simulink model "APFv2_alpha"  (R2025a)
settings: Solver=ode45  StartTime=0.0  StopTime=1  RelTol=1e-3  EnableMultiTasking=on
undefined symbols (not defined in the file): Newton, R_nl, Raphson
libraries: spsDiodeLib x12, spsCurrentMeasurementLib x9, spsSeriesRLCBranchLib x9, spsGroundLib x8, spsVoltageMeasurementLib x5, spsACCurrentSourceLib x3, spsThreePhaseBreakerLib x3, spsThreePhaseSeriesRLCBranchLib x3, spsThreePhaseVIMeasurementLib x2, spsThreePhaseSourceLib x1, powerlib_extras x1, dspfdesign x1
settings Model: Creator=Jawad  LastModifiedBy=SimuVerity Contributors
settings SolverCC: AlgebraicLoopSolver=TrustRegion
settings DataIOCC: LimitDataPoints=on  SaveFormat=Array  SignalLoggingSaveFormat=ModelDataLogs  ReturnWorkspaceOutputs=off
settings OptimizationCC: ExpressionDepthLimit=2147483647.0  LifeSpan=inf
settings DebuggingCC: UnderspecifiedInitializationDetection=Classic  MergeDetectMultiDrivingBlocksExec=none  SolverPrmCheckMsg=warning  FcnCallInpInsideContextMsg=warning  UnconnectedInputMsg=warning  UnconnectedOutputMsg=warning  UnconnectedLineMsg=warning  StateNameClashWarn=warning  SFUnexpectedBacktrackingDiag=warning  SFNoUnconditionalDefaultTransitionDiag=warning  SFExecutionAtInitializationDiag=none  ArithmeticOperatorsInVariantConditions=warning
settings HardwareCC: ProdBitPerPointer=32.0  ProdBitPerSizeT=32.0  ProdBitPerPtrDiffT=32.0  ProdLargestAtomicFloat=None  ProdIntDivRoundTo=Undefined  ProdEndianess=Unspecified  ProdWordSize=32.0  ProdHWDeviceType=32-bit Generic
settings ModelReferenceCC: PropagateSignalLabelsOutOfModel=off
settings SFSimCC: SFSimEcho=off  SimUseLocalCustomCode=off  SimParseCustomCode=off  CustomCodeUndefinedFunction=UseInterfaceOnly
settings RTWCC: RTWUseLocalCustomCode=off  GPUComputeCapability=3.5
settings CodeAppCC: StateflowObjectComments=on
settings GRTTargetCC: TargetLangStandard=C89/C90 (ANSI)  CombineOutputUpdateFcns=off  GRTInterface=on
settings ConfigComp: CovMetricSettings=dw  CovSaveCumulativeToWorkspaceVar=on  CovSaveSingleToWorkspaceVar=on  CovExternalEMLEnable=off

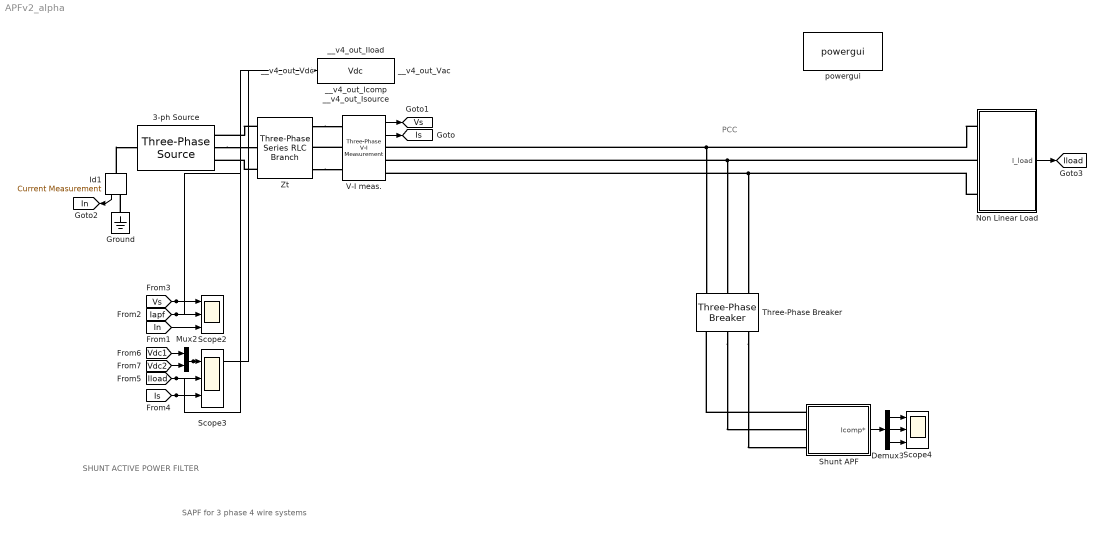
== system APFv2_alpha ==
  note: SHUNT ACTIVE POWER FILTER
  note: PCC
  note: SAPF for 3 phase 4 wire systems
  3-ph Source : spsThreePhaseSourceLib/Three-Phase Source  InternalConnection=Yn  VoltagePhases=off  Voltage=400  PhaseAngle=0  Voltage_phases=[25e3 25e3 25e3]/sqrt(3)  PhaseAngles_phases=[0 -120 +120]  Frequency=50  NonIdealSource=on  SpecifyImpedance=off  Resistance=0.001  Inductance=1e-8  ShortCircuitLevel=100e6  BaseVoltage=25e3  XRratio=7  BusType=swing  Pref=10e3  Qref=0  Prefabc=[10e3, 10e3, 10e3]  Qrefabc=[0, 0, 0]  Qmin=-inf  Qmax=inf
  Demux3 : Demux  Outputs=3
  Ground : spsGroundLib/Ground  LConnTagsString=a
  Id1 : spsCurrentMeasurementLib/Current Measurement  Tag=PoWeRsYsTeMmEaSuReMeNt  PhasorSimulation=off  OutputType=Magnitude  PSBequivalent=0
      settings: AttributesFormatString=\n
  Mux2 : Mux  Inputs=2
  Non Linear Load : Subsystem
  Scope2 : Scope  NumInputPorts=3
      settings: TimeSpan=0.1  ActiveDisplayYMinimum=-350  ActiveDisplayYMaximum=350  DataLoggingMaxPoints=500000  DataLoggingVariableName=Vs_Iapf_Vdc
  Scope3 : Scope  NumInputPorts=3
      settings: TimeSpan=0.1  ActiveDisplayYMinimum=-750  ActiveDisplayYMaximum=2250  DataLoggingMaxPoints=500000  DataLoggingVariableName=Vs_Iapf_Vdc1
  Scope4 : Scope  NumInputPorts=3
      settings: TimeSpan=0.1  ActiveDisplayYMinimum=-250  ActiveDisplayYMaximum=300  DataLoggingMaxPoints=500000  DataLoggingVariableName=Icomp
  Shunt APF : Subsystem
  Three-Phase Breaker : spsThreePhaseBreakerLib/Three-Phase Breaker  InitialState=open  SwitchA=on  SwitchB=on  SwitchC=on  SwitchTimes=0  External=off  BreakerResistance=1e-6  SnubberResistance=1e6  SnubberCapacitance=inf  Measurements=None
  V-I meas. : spsThreePhaseVIMeasurementLib/Three-Phase V-I Measurement  VoltageMeasurement=phase-to-ground  SetLabelV=off  LabelV=Vabc  Vpu=off  VpuLL=off  CurrentMeasurement=yes  SetLabelI=off  LabelI=Iabc  Ipu=off  Pbase=100e6  Vbase=500e3  OutputType=Complex  PhasorSimulation=off  PSBequivalent=0
  Zt : spsThreePhaseSeriesRLCBranchLib/Three-Phase Series RLC Branch  LConnTagsString=A|B|C  RConnTagsString=A|B|C  BranchType=RL  Resistance=0.01  Inductance=1e-6  Capacitance=1e-6  Measurements=None
  __v4_out_Icomp : ToWorkspace  VariableName=Icomp  SaveFormat=Timeseries  SampleTime=-1
  __v4_out_Iload : ToWorkspace  VariableName=Iload  SaveFormat=Timeseries  SampleTime=-1
  __v4_out_Isource : ToWorkspace  VariableName=Isource  SaveFormat=Timeseries  SampleTime=-1
  __v4_out_Vac : ToWorkspace  VariableName=Vac  SaveFormat=Timeseries  SampleTime=-1
  __v4_out_Vdc : ToWorkspace  VariableName=Vdc  SaveFormat=Timeseries  SampleTime=-1
  powergui : spspowerguiLib/powergui  Priority=1  SimulationMode=Discrete  SampleTime=5e-6  frequency=60  Iterations=50  frequencyindice=0  Pbase=100e6  ErrMax=1e-4  UnitsV=kV  UnitsW=MW  buscounter=0  FunctionMessages=off  echomessages=off  EnableUseOfTLC=off  CurrentSourceSwitches=off  DisableSnubberDevices=off  DisableRonSwitches=off  DisableVfSwitches=off  DisplayEquations=off  AutomaticDiscreteSolvers=off  SolverType=Tustin/Backward Euler (TBE)  Interpol=off  ExternalGateDelay=off  methode=off  Ts=100  x0status=blocks  SPID=off  SwTol=0  HookPort=off  NonlinearTolerance=1e-4  nMaxIteration=100  ContinueOnMaxIteration=off  RestoreLinks=warning  ResistiveCurrentMeasurement=off  Frange=[0:2:500]  Ylog=off  Xlog=on  ShowGrid=off  save=off  variable=ZData  structure=comp  ZoomFFT=off  StartTime=0.1  cycles=1  DisplayStyle=2  fundamental=50  FreqAxis=off  MaxFrequency=1000  frequencyindicesteady=1  RmsSteady=1  display=off
  tag scope: Iload=global, In=global, Is=global, Vs=global
  wires:
  Non Linear Load/1(I_load) -> [Iload]
  V-I meas./1 -> [Vs]
  V-I meas./2 -> [Is]
  Demux3/1 -> Scope4/1
  Demux3/2 -> Scope4/2
  Demux3/3 -> Scope4/3
  Shunt APF/1(Icomp*) -> Demux3/1
  [Vs] -> Scope2/1, __v4_out_Vac/1
  [Iapf] -> Scope2/2, __v4_out_Icomp/1
  [Is] -> Scope3/3, __v4_out_Isource/1
  [Iload] -> Scope3/2, __v4_out_Iload/1
  Mux2/1 -> Scope3/1, __v4_out_Vdc/1
  [Vdc1] -> Mux2/1
  [Vdc2] -> Mux2/2
  [In] -> Scope2/3
  Id1/1 -> [In]
  connections:
  Zt/RConn1 -- V-I meas./LConn1
  V-I meas./LConn2 -- Zt/RConn2
  Zt/RConn3 -- V-I meas./LConn3
  Zt/LConn1 -- 3-ph Source/RConn1
  3-ph Source/RConn2 -- Zt/LConn2
  Zt/LConn3 -- 3-ph Source/RConn3
  Non Linear Load/LConn1 -- V-I meas./RConn1 -- Three-Phase Breaker/LConn1
  Non Linear Load/LConn2 -- V-I meas./RConn2 -- Three-Phase Breaker/LConn2
  Non Linear Load/LConn3 -- V-I meas./RConn3 -- Three-Phase Breaker/LConn3
  Shunt APF/LConn1 -- Three-Phase Breaker/RConn1
  Three-Phase Breaker/RConn2 -- Shunt APF/LConn2
  Three-Phase Breaker/RConn3 -- Shunt APF/LConn3
  Id1/LConn1 -- 3-ph Source/LConn1
  Ground/LConn1 -- Id1/RConn1

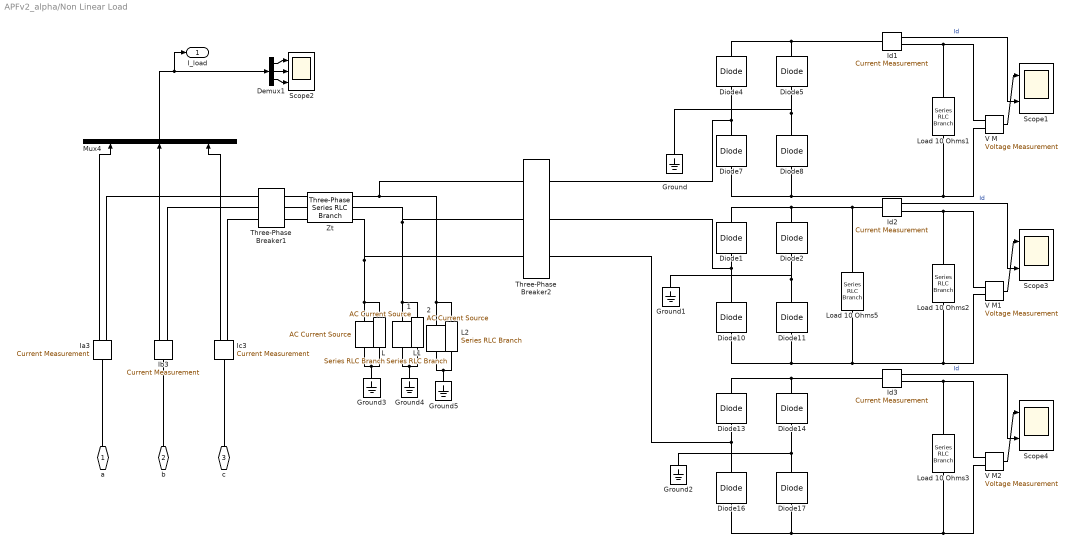
== system APFv2_alpha/Non Linear Load ==
  " " : spsACCurrentSourceLib/AC Current Source  Amplitude=100  Phase=0  Frequency=350  SampleTime=0  Measurements=None
      settings: LibrarySourceBlock=sps_lib/Sources/AC Current Source
  " 1" : spsACCurrentSourceLib/AC Current Source  Amplitude=100  Phase=0  Frequency=250  SampleTime=0  Measurements=None
      settings: LibrarySourceBlock=sps_lib/Sources/AC Current Source
  " 2" : spsACCurrentSourceLib/AC Current Source  Amplitude=100  Phase=0  Frequency=150  SampleTime=0  Measurements=None
      settings: LibrarySourceBlock=sps_lib/Sources/AC Current Source
  Demux1 : Demux  Outputs=3
  Diode{1..2,4..5,7..8,10..11,13..14,16..17} (12 alike) : spsDiodeLib/Diode  Ron=1e-1  Lon=0  Vf=0.8  IC=0  UseSnubber=off  Rs=1000  Cs=0.1e-6  Measurements=off
      settings: AttributesFormatString=\n
  Ground{,1..5} (6 alike) : spsGroundLib/Ground  LConnTagsString=a
  Ia3 : spsCurrentMeasurementLib/Current Measurement  PhasorSimulation=off  OutputType=Complex  PSBequivalent=0
  Ib3 : spsCurrentMeasurementLib/Current Measurement  PhasorSimulation=off  OutputType=Complex  PSBequivalent=0
  Ic3 : spsCurrentMeasurementLib/Current Measurement  PhasorSimulation=off  OutputType=Complex  PSBequivalent=0
  Id1 : spsCurrentMeasurementLib/Current Measurement  Tag=PoWeRsYsTeMmEaSuReMeNt  PhasorSimulation=off  OutputType=Magnitude  PSBequivalent=0
      settings: AttributesFormatString=\n
  Id2 : spsCurrentMeasurementLib/Current Measurement  Tag=PoWeRsYsTeMmEaSuReMeNt  PhasorSimulation=off  OutputType=Magnitude  PSBequivalent=0
      settings: AttributesFormatString=\n
  Id3 : spsCurrentMeasurementLib/Current Measurement  Tag=PoWeRsYsTeMmEaSuReMeNt  PhasorSimulation=off  OutputType=Magnitude  PSBequivalent=0
      settings: AttributesFormatString=\n
  L : spsSeriesRLCBranchLib/Series RLC Branch  LConnTagsString=__new0  RConnTagsString=__new0  BranchType=R  Resistance=1000000000  Inductance=8e-3  SetiL0=off  InitialCurrent=0  Capacitance=[]  Setx0=off  InitialVoltage=0  Measurements=None
  L1 : spsSeriesRLCBranchLib/Series RLC Branch  LConnTagsString=__new0  RConnTagsString=__new0  BranchType=R  Resistance=1000000000  Inductance=8e-3  SetiL0=off  InitialCurrent=0  Capacitance=[]  Setx0=off  InitialVoltage=0  Measurements=None
  L2 : spsSeriesRLCBranchLib/Series RLC Branch  LConnTagsString=__new0  RConnTagsString=__new0  BranchType=R  Resistance=1000000000  Inductance=8e-3  SetiL0=off  InitialCurrent=0  Capacitance=[]  Setx0=off  InitialVoltage=0  Measurements=None
  Load 10 Ohms1 : spsSeriesRLCBranchLib/Series RLC Branch  LConnTagsString=__new0  RConnTagsString=__new0  BranchType=RL  Resistance=R_nl  Inductance=1e-3  SetiL0=off  InitialCurrent=0  Capacitance=[]  Setx0=off  InitialVoltage=0  Measurements=None
  Load 10 Ohms2 : spsSeriesRLCBranchLib/Series RLC Branch  LConnTagsString=__new0  RConnTagsString=__new0  BranchType=R  Resistance=4  Inductance=8e-3  SetiL0=off  InitialCurrent=0  Capacitance=[]  Setx0=off  InitialVoltage=0  Measurements=None
  Load 10 Ohms3 : spsSeriesRLCBranchLib/Series RLC Branch  LConnTagsString=__new0  RConnTagsString=__new0  BranchType=R  Resistance=3  Inductance=3e-3  SetiL0=off  InitialCurrent=0  Capacitance=[]  Setx0=off  InitialVoltage=0  Measurements=None
  Load 10 Ohms5 : spsSeriesRLCBranchLib/Series RLC Branch  LConnTagsString=__new0  RConnTagsString=__new0  BranchType=C  Resistance=20  Inductance=20e-3  SetiL0=off  InitialCurrent=0  Capacitance=50e-6  Setx0=off  InitialVoltage=0  Measurements=None
  Mux4 : Mux  Inputs=3
  Scope1 : Scope  NumInputPorts=2
      settings: TimeSpan=0.1  ActiveDisplayYMinimum=-10.5  ActiveDisplayYMaximum=-1.5  DataLoggingSaveFormat=Structure
  Scope2 : Scope  NumInputPorts=3
      settings: TimeSpan=0.1  ActiveDisplayYMinimum=-70  ActiveDisplayYMaximum=80  DataLoggingMaxPoints=500000  DataLoggingVariableName=i_load
  Scope3 : Scope  NumInputPorts=2
      settings: TimeSpan=0.1  ActiveDisplayYMinimum=475  ActiveDisplayYMaximum=555  DataLoggingSaveFormat=Structure
  Scope4 : Scope  NumInputPorts=2
      settings: TimeSpan=0.1  ActiveDisplayYMinimum=475  ActiveDisplayYMaximum=555  DataLoggingVariableName=ScopeData2  DataLoggingSaveFormat=Structure
  Three-Phase Breaker1 : spsThreePhaseBreakerLib/Three-Phase Breaker  InitialState=open  SwitchA=on  SwitchB=on  SwitchC=on  SwitchTimes=0  External=off  BreakerResistance=1e-5  SnubberResistance=1e6  SnubberCapacitance=inf  Measurements=None
  Three-Phase Breaker2 : spsThreePhaseBreakerLib/Three-Phase Breaker  InitialState=open  SwitchA=on  SwitchB=on  SwitchC=on  SwitchTimes=0  External=off  BreakerResistance=1e-5  SnubberResistance=1e6  SnubberCapacitance=inf  Measurements=None
  V M : spsVoltageMeasurementLib/Voltage Measurement  PhasorSimulation=off  OutputType=Complex  PSBequivalent=0
  V M1 : spsVoltageMeasurementLib/Voltage Measurement  PhasorSimulation=off  OutputType=Complex  PSBequivalent=0
  V M2 : spsVoltageMeasurementLib/Voltage Measurement  PhasorSimulation=off  OutputType=Complex  PSBequivalent=0
  Zt : spsThreePhaseSeriesRLCBranchLib/Three-Phase Series RLC Branch  LConnTagsString=A|B|C  RConnTagsString=A|B|C  BranchType=RL  Resistance=0.00001  Inductance=1e-4  Capacitance=1e-6  Measurements=None
  a : PMIOPort  Side=Left
  b : PMIOPort  Port=2  Side=Left
  c : PMIOPort  Port=3  Side=Left
  I_load : Outport
  wires:
  Mux4/1 -> I_load/1, Demux1/1
  Demux1/2 -> Scope2/2
  Demux1/3 -> Scope2/3
  Demux1/1 -> Scope2/1
  Ic3/1 -> Mux4/3
  Ib3/1 -> Mux4/2
  Ia3/1 -> Mux4/1
  V M/1 -> Scope1/1
  Id1/1 -> Scope1/2  "Id"
  V M1/1 -> Scope3/1
  Id2/1 -> Scope3/2  "Id"
  V M2/1 -> Scope4/1
  Id3/1 -> Scope4/2  "Id"
  connections:
  Ia3/LConn1 -- a/RConn1
  Ib3/LConn1 -- b/RConn1
  Three-Phase Breaker1/LConn3 -- Ic3/RConn1
  Three-Phase Breaker1/LConn2 -- Ib3/RConn1
  Ia3/RConn1 -- Three-Phase Breaker1/LConn1
  c/RConn1 -- Ic3/LConn1
  Zt/LConn1 -- Three-Phase Breaker1/RConn1
  Three-Phase Breaker1/RConn2 -- Zt/LConn2
  Zt/LConn3 -- Three-Phase Breaker1/RConn3
  Id1/LConn1 -- Diode4/RConn1 -- Diode5/RConn1
  V M/LConn1 -- Load 10 Ohms1/LConn1 -- Id1/RConn1
  Diode7/LConn1 -- Diode8/LConn1 -- V M/LConn2 -- Load 10 Ohms1/RConn1
  Ground/LConn1 -- Diode5/LConn1 -- Diode8/RConn1
  Load 10 Ohms5/LConn1 -- Id2/LConn1 -- Diode1/RConn1 -- Diode2/RConn1
  V M1/LConn1 -- Load 10 Ohms2/LConn1 -- Id2/RConn1
  V M1/LConn2 -- Load 10 Ohms2/RConn1 -- Diode10/LConn1 -- Diode11/LConn1 -- Load 10 Ohms5/RConn1
  Zt/RConn2 -- " 1"/LConn1 -- L1/LConn1 -- Three-Phase Breaker2/LConn2
  Ground1/LConn1 -- Diode2/LConn1 -- Diode11/RConn1
  Id3/LConn1 -- Diode13/RConn1 -- Diode14/RConn1
  V M2/LConn1 -- Load 10 Ohms3/LConn1 -- Id3/RConn1
  V M2/LConn2 -- Load 10 Ohms3/RConn1 -- Diode16/LConn1 -- Diode17/LConn1
  Diode13/LConn1 -- Diode16/RConn1 -- Three-Phase Breaker2/RConn3
  Diode14/LConn1 -- Diode17/RConn1 -- Ground2/LConn1
  " "/RConn1 -- L/RConn1 -- Ground3/LConn1
  Ground4/LConn1 -- " 1"/RConn1 -- L1/RConn1
  Ground5/LConn1 -- " 2"/RConn1 -- L2/RConn1
  Zt/RConn1 -- " 2"/LConn1 -- L2/LConn1 -- Three-Phase Breaker2/LConn1
  Diode7/RConn1 -- Diode4/LConn1 -- Three-Phase Breaker2/RConn1
  " "/LConn1 -- L/LConn1 -- Zt/RConn3 -- Three-Phase Breaker2/LConn3
  Diode1/LConn1 -- Diode10/RConn1 -- Three-Phase Breaker2/RConn2

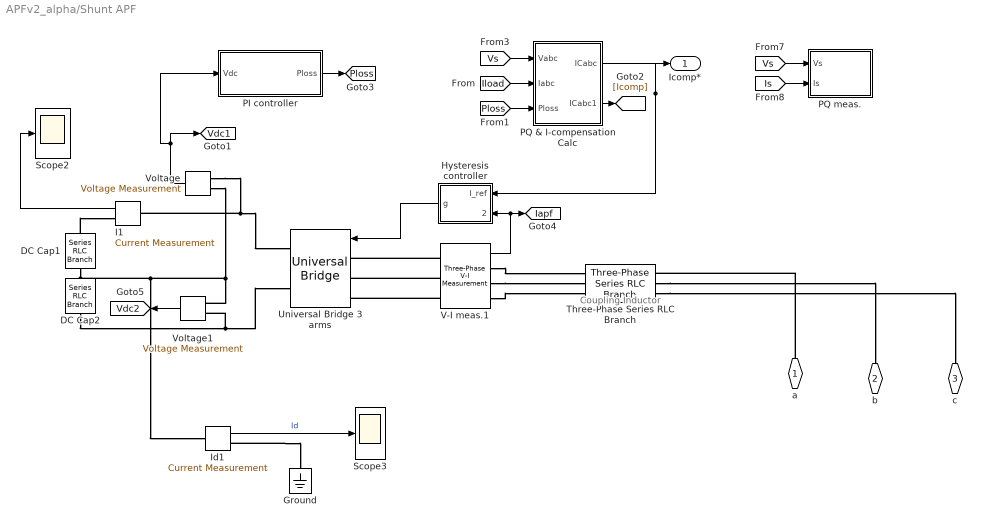
== system APFv2_alpha/Shunt APF ==
  note: Coupling Inductor
  DC Cap1 : spsSeriesRLCBranchLib/Series RLC Branch  LConnTagsString=__new0  RConnTagsString=__new0  BranchType=C  Resistance=1  Inductance=1e-3  SetiL0=off  InitialCurrent=0  Capacitance=400e-6  Setx0=off  InitialVoltage=400  Measurements=None
  DC Cap2 : spsSeriesRLCBranchLib/Series RLC Branch  LConnTagsString=__new0  RConnTagsString=__new0  BranchType=C  Resistance=1  Inductance=5e-3  SetiL0=off  InitialCurrent=0  Capacitance=400e-6  Setx0=off  InitialVoltage=400  Measurements=None
  Ground : spsGroundLib/Ground  LConnTagsString=a
  Hysteresis controller : Subsystem
  I1 : spsCurrentMeasurementLib/Current Measurement  Tag=PoWeRsYsTeMmEaSuReMeNt  PhasorSimulation=off  OutputType=Magnitude  PSBequivalent=0
      settings: AttributesFormatString=\n
  Id1 : spsCurrentMeasurementLib/Current Measurement  Tag=PoWeRsYsTeMmEaSuReMeNt  PhasorSimulation=off  OutputType=Magnitude  PSBequivalent=0
      settings: AttributesFormatString=\n
  PI controller : Subsystem
  PQ & I-compensation Calc : Subsystem
  PQ meas. : Subsystem
  Scope2 : Scope
      settings: TimeSpan=0.1  ActiveDisplayYMinimum=-110  ActiveDisplayYMaximum=100  DataLoggingMaxPoints=500000  DataLoggingVariableName=psb3phPWM1_str4
  Scope3 : Scope
      settings: TimeSpan=0.1  ActiveDisplayYMinimum=-1  ActiveDisplayYMaximum=1  DataLoggingVariableName=ScopeData3  DataLoggingSaveFormat=Structure
  Three-Phase Series RLC Branch : spsThreePhaseSeriesRLCBranchLib/Three-Phase Series RLC Branch  LConnTagsString=A|B|C  RConnTagsString=A|B|C  BranchType=L  Resistance=1e9  Inductance=2e-3  Capacitance=.2e-3  Measurements=None
  Universal Bridge 3 arms : spsUniversalBridgeLib/Universal Bridge  Arms=3  SnubberResistance=10000  SnubberCapacitance=inf  Device=IGBT / Diodes  Ron=1e-4  Lon=0  ForwardVoltages="[  1  1  ]"  ForwardVoltage=.8  GTOparameters=[ 10e-6 , 20e-6 ]  IGBTparameters=[ 1e-6 , 2e-6 ]  Measurements=None  Measurements_2=None  converterType=Rectifier
      settings: AttributesFormatString=\n
  V-I meas.1 : spsThreePhaseVIMeasurementLib/Three-Phase V-I Measurement  VoltageMeasurement=phase-to-ground  SetLabelV=on  LabelV=Vabc  Vpu=off  VpuLL=off  CurrentMeasurement=yes  SetLabelI=off  LabelI=Iabc  Ipu=off  Pbase=100e6  Vbase=500e3  OutputType=Complex  PhasorSimulation=off  PSBequivalent=0
  Voltage : spsVoltageMeasurementLib/Voltage Measurement  PhasorSimulation=off  OutputType=Complex  PSBequivalent=0
  Voltage1 : spsVoltageMeasurementLib/Voltage Measurement  PhasorSimulation=off  OutputType=Complex  PSBequivalent=0
  a : PMIOPort  Side=Left
  b : PMIOPort  Port=2  Side=Left
  c : PMIOPort  Port=3  Side=Left
  Icomp* : Outport
  tag scope: Iapf=global, Ploss=global, Vdc1=global, Vdc2=global
  wires:
  [Iload] -> PQ & I-compensation Calc/2(Iabc)
  V-I meas.1/1 -> Hysteresis controller/2(I_meas), [Iapf]
  PQ & I-compensation Calc/1(ICabc) -> Hysteresis controller/1(I_ref), Icomp*/1
  [Vs] -> PQ & I-compensation Calc/1(Vabc)
  PQ & I-compensation Calc/2(ICabc1) -> [Icomp]
  PI controller/1(Ploss) -> [Ploss]
  [Ploss] -> PQ & I-compensation Calc/3(Ploss)
  [Vs] -> PQ meas./1(Vs)
  [Is] -> PQ meas./2(Is)
  Voltage/1 -> [Vdc1], PI controller/1(Vdc)
  I1/1 -> Scope2/1
  Hysteresis controller/1(g) -> Universal Bridge 3 arms/1
  Voltage1/1 -> [Vdc2]
  Id1/1 -> Scope3/1  "Id"
  connections:
  Voltage/LConn1 -- Universal Bridge 3 arms/RConn1 -- I1/LConn1
  V-I meas.1/LConn1 -- Universal Bridge 3 arms/LConn1
  V-I meas.1/LConn2 -- Universal Bridge 3 arms/LConn2
  V-I meas.1/RConn3 -- Three-Phase Series RLC Branch/LConn3
  V-I meas.1/RConn2 -- Three-Phase Series RLC Branch/LConn2
  V-I meas.1/LConn3 -- Universal Bridge 3 arms/LConn3
  DC Cap2/RConn1 -- Universal Bridge 3 arms/RConn2 -- Voltage1/LConn2
  V-I meas.1/RConn1 -- Three-Phase Series RLC Branch/LConn1
  a/RConn1 -- Three-Phase Series RLC Branch/RConn1
  Three-Phase Series RLC Branch/RConn2 -- b/RConn1
  Three-Phase Series RLC Branch/RConn3 -- c/RConn1
  DC Cap1/LConn1 -- I1/RConn1
  Voltage/LConn2 -- Voltage1/LConn1 -- DC Cap1/RConn1 -- DC Cap2/LConn1 -- Id1/LConn1
  Id1/RConn1 -- Ground/LConn1

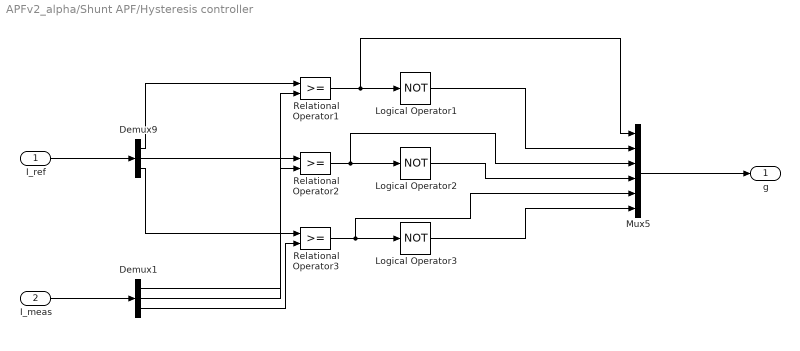
== system APFv2_alpha/Shunt APF/Hysteresis controller ==
  I_ref : Inport
  I_meas : Inport  Port=2
  Demux1 : Demux  Outputs=3
  Demux9 : Demux  Outputs=3
  Logical Operator1 : Logic  Operator=NOT  AllPortsSameDT=off  OutDataTypeStr=boolean
  Logical Operator2 : Logic  Operator=NOT  AllPortsSameDT=off  OutDataTypeStr=boolean
  Logical Operator3 : Logic  Operator=NOT  AllPortsSameDT=off  OutDataTypeStr=boolean
  Mux5 : Mux  Inputs=6
  Relational Operator1 : RelationalOperator  OutDataTypeStr=boolean  InputSameDT=off
  Relational Operator2 : RelationalOperator  OutDataTypeStr=boolean  InputSameDT=off
  Relational Operator3 : RelationalOperator  OutDataTypeStr=boolean  InputSameDT=off
  g : Outport
  wires:
  Relational Operator1/1 -> Logical Operator1/1, Mux5/1
  Relational Operator2/1 -> Logical Operator2/1, Mux5/3
  Relational Operator3/1 -> Logical Operator3/1, Mux5/5
  Demux9/1 -> Relational Operator1/1
  Demux9/3 -> Relational Operator3/1
  Logical Operator1/1 -> Mux5/2
  Logical Operator2/1 -> Mux5/4
  Logical Operator3/1 -> Mux5/6
  Mux5/1 -> g/1
  Demux9/2 -> Relational Operator2/1
  Demux1/1 -> Relational Operator1/2
  Demux1/2 -> Relational Operator2/2
  Demux1/3 -> Relational Operator3/2
  I_ref/1 -> Demux9/1
  I_meas/1 -> Demux1/1

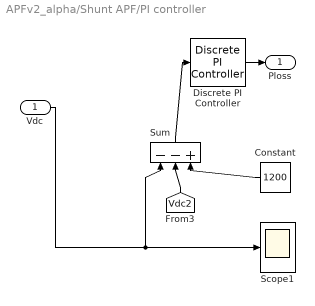
== system APFv2_alpha/Shunt APF/PI controller ==
  Vdc : Inport
  Constant : Constant  Value=1200
  Discrete PI Controller : powerlib_extras/Discrete  Control Blocks/Discrete PI Controller  Kp=0.5  Ki=1  Par_Limits=[1e6 -1e6]  Init=0  Ts=5e-6
  Scope1 : Scope
      settings: TimeSpan=0.1  ActiveDisplayYMinimum=-1  ActiveDisplayYMaximum=1  DataLoggingMaxPoints=500000  DataLoggingVariableName=psb3phPWM1_str1
  Sum : Sum  Inputs=|--+
  Ploss : Outport
  wires:
  Sum/1 -> Discrete PI Controller/1
  Discrete PI Controller/1 -> Ploss/1
  Vdc/1 -> Scope1/1, Sum/1
  [Vdc2] -> Sum/2
  Constant/1 -> Sum/3

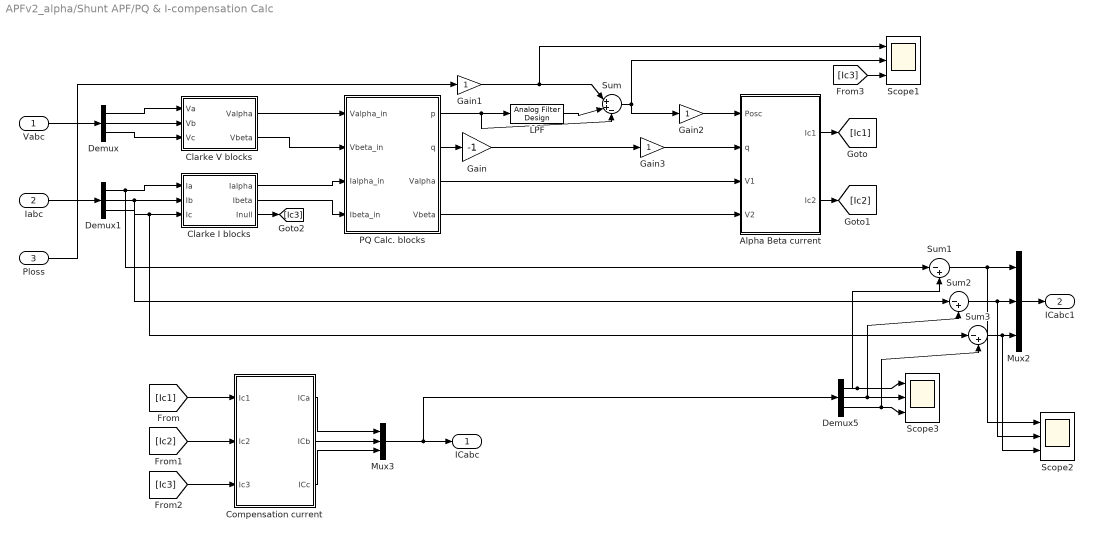
== system APFv2_alpha/Shunt APF/PQ & I-compensation Calc ==
  Vabc : Inport
  Iabc : Inport  Port=2
  Ploss : Inport  Port=3
  Alpha Beta current : MATLAB Function  TreatAsAtomicUnit=on
  Clarke I blocks : Subsystem
  Clarke V blocks : Subsystem
  Compensation current : MATLAB Function  TreatAsAtomicUnit=on
  Demux : Demux  Outputs=3
  Demux1 : Demux  Outputs=3
  Demux5 : Demux  Outputs=3
  Gain : Gain  Gain=-1
  Gain1 : Gain
  Gain2 : Gain
  Gain3 : Gain
  LPF : dspfdesign/Analog Filter Design  method=Butterworth  filttype=Lowpass  N=5  Wlo=2*pi*50  Whi=80  Rp=2  Rs=40
  Mux2 : Mux  Inputs=3
  Mux3 : Mux  Inputs=3
  PQ Calc. blocks : Subsystem
  Scope1 : Scope  NumInputPorts=3
      settings: TimeSpan=0.1  ActiveDisplayYMinimum=4700  ActiveDisplayYMaximum=5700  DataLoggingMaxPoints=500000  DataLoggingVariableName=psb3phPWM1_str9
  Scope2 : Scope  NumInputPorts=3
      settings: TimeSpan=0.1  ActiveDisplayYMinimum=-3.55  ActiveDisplayYMaximum=-2.8  DataLoggingMaxPoints=500000  DataLoggingVariableName=comp_plus_load
  Scope3 : Scope  NumInputPorts=3
      settings: TimeSpan=0.1  ActiveDisplayYMinimum=-1  ActiveDisplayYMaximum=1  DataLoggingMaxPoints=500000  DataLoggingVariableName=comp
  Sum : Sum  Inputs=|++-
  Sum1 : Sum  Inputs=|-+
  Sum2 : Sum  Inputs=|-+
  Sum3 : Sum  Inputs=|-+
  ICabc : Outport
  ICabc1 : Outport  Port=2
  wires:
  Iabc/1 -> Demux1/1
  Vabc/1 -> Demux/1
  [Ic1] -> Compensation current/1(Ic1)
  [Ic2] -> Compensation current/2(Ic2)
  Compensation current/1(ICa) -> Mux3/1
  Compensation current/2(ICb) -> Mux3/2
  Compensation current/3(ICc) -> Mux3/3
  Clarke V blocks/1(Valpha) -> PQ Calc. blocks/1(Valpha_in)
  Clarke V blocks/2(Vbeta) -> PQ Calc. blocks/2(Vbeta_in)
  Clarke I blocks/1(Ialpha) -> PQ Calc. blocks/3(Ialpha_in)
  PQ Calc. blocks/2(q) -> Gain/1
  PQ Calc. blocks/1(p) -> LPF/1, Sum/3
  Gain/1 -> Gain3/1
  PQ Calc. blocks/3(Valpha) -> Alpha Beta current/3(V1)
  Alpha Beta current/1(Ic1) -> [Ic1]
  Alpha Beta current/2(Ic2) -> [Ic2]
  Clarke I blocks/2(Ibeta) -> PQ Calc. blocks/4(Ibeta_in)
  PQ Calc. blocks/4(Vbeta) -> Alpha Beta current/4(V2)
  Demux/1 -> Clarke V blocks/1(Va)
  Demux/2 -> Clarke V blocks/2(Vb)
  Demux/3 -> Clarke V blocks/3(Vc)
  Demux1/1 -> Sum1/1, Clarke I blocks/1(Ia)
  Demux1/2 -> Sum2/1, Clarke I blocks/2(Ib)
  Demux1/3 -> Sum3/1, Clarke I blocks/3(Ic)
  LPF/1 -> Sum/2
  Sum/1 -> Scope1/2, Gain2/1
  Gain1/1 -> Sum/1, Scope1/1
  Mux3/1 -> ICabc/1, Demux5/1
  Demux5/1 -> Scope3/1, Sum1/2
  Demux5/2 -> Scope3/2, Sum2/2
  Demux5/3 -> Scope3/3, Sum3/2
  Ploss/1 -> Gain1/1
  Sum1/1 -> Mux2/1, Scope2/1
  Sum2/1 -> Mux2/2, Scope2/2
  Sum3/1 -> Mux2/3, Scope2/3
  Mux2/1 -> ICabc1/1
  Gain2/1 -> Alpha Beta current/1(Posc)
  Gain3/1 -> Alpha Beta current/2(q)
  Clarke I blocks/3(Inull) -> [Ic3]
  [Ic3] -> Compensation current/3(Ic3)
  [Ic3] -> Scope1/3

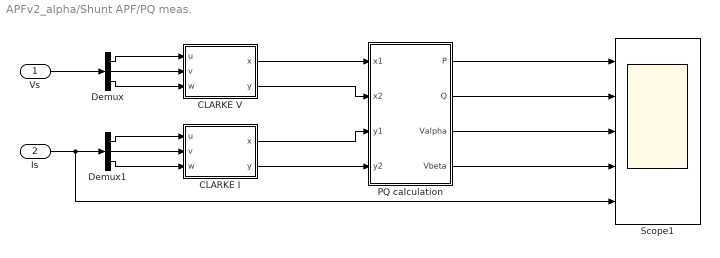
== system APFv2_alpha/Shunt APF/PQ meas. ==
  Vs : Inport
  Is : Inport  Port=2
  CLARKE I : MATLAB Function  TreatAsAtomicUnit=on
  CLARKE V : MATLAB Function  TreatAsAtomicUnit=on
  Demux : Demux  Outputs=3
  Demux1 : Demux  Outputs=3
  PQ calculation : MATLAB Function  TreatAsAtomicUnit=on
  Scope1 : Scope  NumInputPorts=5
      settings: TimeSpan=0.1  ActiveDisplayYMinimum=0  ActiveDisplayYMaximum=70000  DataLoggingMaxPoints=500000  DataLoggingVariableName=psb3phPWM1_str
  wires:
  CLARKE V/1(x) -> PQ calculation/1(x1)
  CLARKE V/2(y) -> PQ calculation/2(x2)
  CLARKE I/1(x) -> PQ calculation/3(y1)
  CLARKE I/2(y) -> PQ calculation/4(y2)
  Demux/1 -> CLARKE V/1(u)
  Demux/2 -> CLARKE V/2(v)
  Demux/3 -> CLARKE V/3(w)
  Demux1/1 -> CLARKE I/1(u)
  Demux1/2 -> CLARKE I/2(v)
  Demux1/3 -> CLARKE I/3(w)
  Vs/1 -> Demux/1
  Is/1 -> Demux1/1, Scope1/5
  PQ calculation/1(P) -> Scope1/1
  PQ calculation/2(Q) -> Scope1/2
  PQ calculation/3(Valpha) -> Scope1/3
  PQ calculation/4(Vbeta) -> Scope1/4

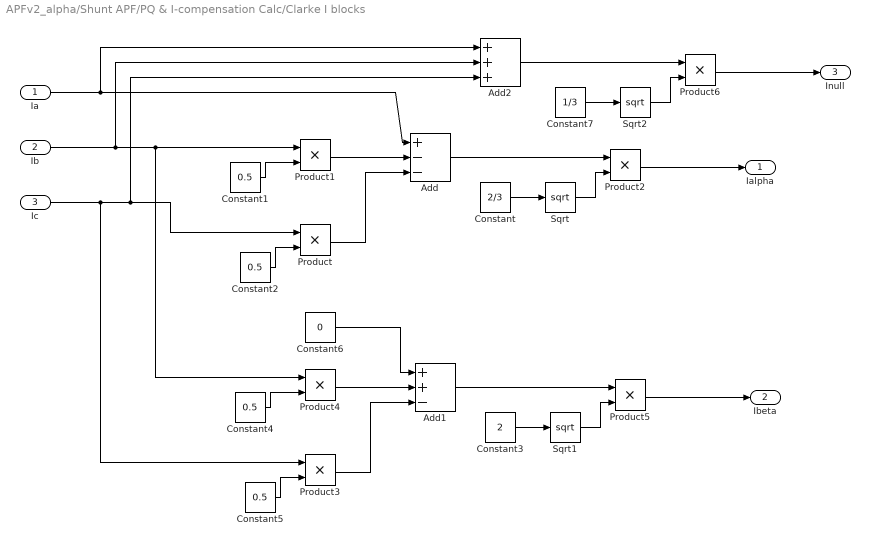
== system APFv2_alpha/Shunt APF/PQ & I-compensation Calc/Clarke I blocks ==
  Ia : Inport
  Ib : Inport  Port=2
  Ic : Inport  Port=3
  Add : Sum  Inputs=+--
  Add1 : Sum  Inputs=++-
  Add2 : Sum  Inputs=+++
  Constant : Constant  Value=2/3
  Constant{1..2,4..5} (4 alike) : Constant  Value=0.5
  Constant3 : Constant  Value=2
  Constant6 : Constant  Value=0
  Constant7 : Constant  Value=1/3
  Product{,1..6} (7 alike) : Product  RndMeth=Zero
  Sqrt : Sqrt  AlgorithmType=Newton-Raphson
  Sqrt1 : Sqrt  AlgorithmType=Newton-Raphson
  Sqrt2 : Sqrt  AlgorithmType=Newton-Raphson
  Ialpha : Outport
  Ibeta : Outport  Port=2
  Inull : Outport  Port=3
  wires:
  Sqrt1/1 -> Product5/2
  Constant3/1 -> Sqrt1/1
  Product5/1 -> Ibeta/1
  Add1/1 -> Product5/1
  Product3/1 -> Add1/3
  Constant5/1 -> Product3/2
  Product4/1 -> Add1/2
  Constant4/1 -> Product4/2
  Constant6/1 -> Add1/1
  Ic/1 -> Product3/1, Product/1, Add2/3
  Sqrt/1 -> Product2/2
  Constant/1 -> Sqrt/1
  Product2/1 -> Ialpha/1
  Add/1 -> Product2/1
  Product/1 -> Add/3
  Constant2/1 -> Product/2
  Product1/1 -> Add/2
  Constant1/1 -> Product1/2
  Ib/1 -> Product4/1, Product1/1, Add2/2
  Ia/1 -> Add/1, Add2/1
  Sqrt2/1 -> Product6/2
  Constant7/1 -> Sqrt2/1
  Product6/1 -> Inull/1
  Add2/1 -> Product6/1

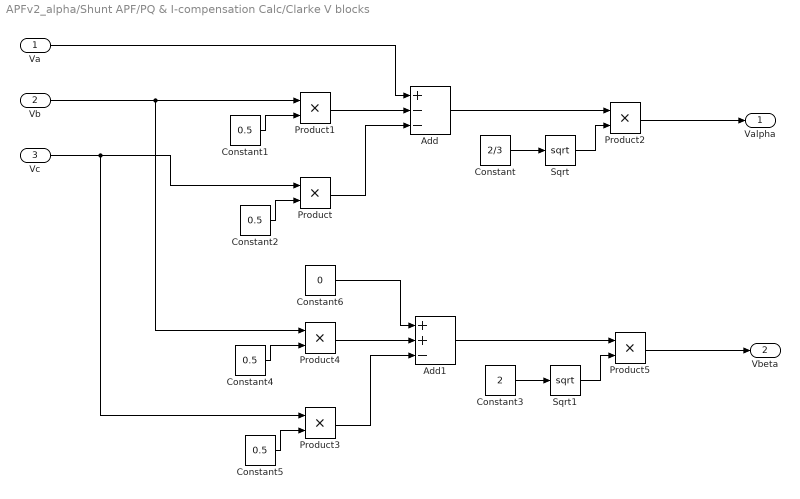
== system APFv2_alpha/Shunt APF/PQ & I-compensation Calc/Clarke V blocks ==
  Va : Inport
  Vb : Inport  Port=2
  Vc : Inport  Port=3
  Add : Sum  Inputs=+--
  Add1 : Sum  Inputs=++-
  Constant : Constant  Value=2/3
  Constant{1..2,4..5} (4 alike) : Constant  Value=0.5
  Constant3 : Constant  Value=2
  Constant6 : Constant  Value=0
  Product{,1..5} (6 alike) : Product  RndMeth=Zero
  Sqrt : Sqrt  AlgorithmType=Newton-Raphson
  Sqrt1 : Sqrt  AlgorithmType=Newton-Raphson
  Valpha : Outport
  Vbeta : Outport  Port=2
  wires:
  Va/1 -> Add/1
  Vb/1 -> Product1/1, Product4/1
  Constant1/1 -> Product1/2
  Product1/1 -> Add/2
  Constant2/1 -> Product/2
  Product/1 -> Add/3
  Add/1 -> Product2/1
  Product2/1 -> Valpha/1
  Constant/1 -> Sqrt/1
  Sqrt/1 -> Product2/2
  Vc/1 -> Product/1, Product3/1
  Constant6/1 -> Add1/1
  Constant4/1 -> Product4/2
  Product4/1 -> Add1/2
  Constant5/1 -> Product3/2
  Product3/1 -> Add1/3
  Add1/1 -> Product5/1
  Product5/1 -> Vbeta/1
  Constant3/1 -> Sqrt1/1
  Sqrt1/1 -> Product5/2

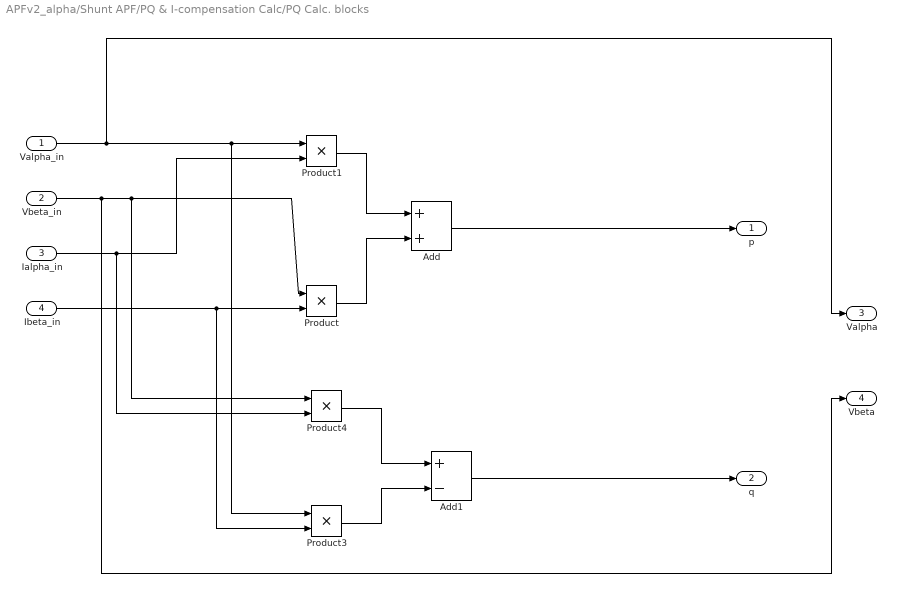
== system APFv2_alpha/Shunt APF/PQ & I-compensation Calc/PQ Calc. blocks ==
  Valpha_in : Inport
  Vbeta_in : Inport  Port=2
  Ialpha_in : Inport  Port=3
  Ibeta_in : Inport  Port=4
  Add : Sum
  Add1 : Sum  Inputs=+-
  Product{,1,3..4} (4 alike) : Product  RndMeth=Zero
  p : Outport
  q : Outport  Port=2
  Valpha : Outport  Port=3
  Vbeta : Outport  Port=4
  wires:
  Valpha_in/1 -> Product1/1, Product3/1, Valpha/1
  Ialpha_in/1 -> Product1/2, Product4/2
  Vbeta_in/1 -> Product/1, Product4/1, Vbeta/1
  Ibeta_in/1 -> Product/2, Product3/2
  Product1/1 -> Add/1
  Product/1 -> Add/2
  Product4/1 -> Add1/1
  Product3/1 -> Add1/2
  Add1/1 -> q/1
  Add/1 -> p/1

== matlab function APFv2_alpha/Shunt APF/PQ & I-compensation Calc/Compensation current ==
  data: Ic1 input; ICa output; Ic2 input; ICb output; ICc output; Ic3 input
function [ICa,ICb,ICc] = Ical(Ic1,Ic2,Ic3)
%#em1

ICa = sqrt(2/3)*(Ic1+(0.7072*Ic3));
ICb = sqrt(2/3)*((-0.5*Ic1)+((sqrt(3)/2)*Ic2)+(0.7072*Ic3));
ICc = sqrt(2/3)*((-0.5*Ic1)-((sqrt(3)/2)*Ic2)+(0.7072*Ic3));

== matlab function APFv2_alpha/Shunt APF/PQ & I-compensation Calc/Alpha Beta current ==
  data: Posc input; Ic1 output; q input; V1 input; Ic2 output; V2 input
function [Ic1,Ic2] = ICOM(Posc,q,V1,V2)
%#em1

Ic1 = (-1/(V1^2 + V2^2))*((Posc*V1)+(q*V2));
Ic2 = (-1/(V1^2 + V2^2))*((Posc*V2)-(q*V1));

== matlab function APFv2_alpha/Shunt APF/PQ meas./CLARKE I ==
  data: u input; x output; v input; w input; y output
function [x,y] = ICT(u,v,w)
%#em1

x = sqrt(2/3)*(u-(0.5*v)-(0.5*w));
y = sqrt(2)*(0+(0.5*v)-(0.5*w));

== matlab function APFv2_alpha/Shunt APF/PQ meas./CLARKE V ==
  data: u input; x output; v input; w input; y output
function [x,y] = VCT(u,v,w)
%#em1

x = sqrt(2/3)*(u-(0.5*v)-(0.5*w));
y = sqrt(2)*(0+(0.5*v)-(0.5*w));

== matlab function APFv2_alpha/Shunt APF/PQ meas./PQ calculation ==
  data: x1 input; P output; Q output; x2 input; y1 input; y2 input; Valpha output; Vbeta output
function [P,Q,Valpha,Vbeta] = PQ(x1,x2,y1,y2)
%#em1

P = (x1*y1)+(x2*y2);
Q = (x2*y1)-(x1*y2);
Valpha = x1;
Vbeta = x2;
